simulink model "RobustFormationControl_FractionalModel_under_Dis"  (R2023a)
settings: Solver=ode3  StartTime=0.0  StopTime=30  FixedStep=0.0001  RelTol=1e-3
InitFcn:
  | % close all;
  | % clear all;
  | % clc;
  | % System & Qaudrotor Parameters
  | %==============================
  | m = 0.486;                                         % Quadrotor Mass ( kg )
  | 
  | L = 0.25;                                         % Length of the arm ( m )
  | % L = 0.25;                                         % Length of the arm ( m )
  | 
  | Ixx = 4.856e-03; Iyy = 4.856e-03; Izz = 8.801e-03; % The moments of inertia around x,y and z axes respectively ( kg.m^2 )
  | % Ixx = 3.8278e-03; Iyy = 3.8278e-03; Izz = 7.6566e-03; % The moments of inertia around x,y and z axes respectively ( kg.m^2 )
  | 
  | Jr = 2.8385e-5;                                            % The inertia moment of rotor ( kg.m^2 )
  | % Jr = 0;
  | 
  | % Kx=5.5670e-4;
  | % Ky=5.5670e-4;
  | % Kz=6.3540e-4;
  | % kx=0.032;
  | % ky=0.032;
  | % kz=0.048;
  | Kfx = 5.5670e-4; Kfy = 5.5670e-4; Kfz = 6.3540e-4;% The Rotational drag cofficients ( N/rad/s )
  | 
  | % Ktx = 0.032; Kty = 0.032; Ktz = 0.048;               % The linear drag coefficients in x, y, z respectively ( N/m/s )
  | Ktx = 5.5670e-4; Kty =5.5670e-4; Ktz = 6.3540e-4;               % The linear drag coefficients in x, y, z respectively ( N/m/s )
  | 
  | b = 2.923e-05;                                      % The lift coefficient
  | % b = 2.9842e-05;                                      % The lift coefficient
  | 
  | d = 1.12e-06;                                       % The drag coefficient
  | % d = 3.2320e-07;                                       % The drag coefficient
  | 
  | g = 9.81;                                          % The acceleration due to gravity ( m/s^2 )
  | 
  | %-------- The Coefficients of Non-linear Equations of Quadrotor ( Page 11) -------
  | %--------------------------------------------------------------------------------
  | % Rotational Equations
  | %=====================
  | % Coefficients in ( eq1 ) >>..
  | a1 = (Iyy - Izz)/Ixx;
  | b1 = - Jr/Ixx;
  | c1 = - Kfx/Ixx;
  | d1 = L/Ixx;
  | 
  | % Coefficients in ( eq2 ) >>..
  | a2 = (Izz - Ixx)/Iyy;
  | b2 = Jr/Iyy;
  | c2 = - Kfy/Iyy;
  | d2 = L/Iyy;
  | 
  | % Coefficients in ( eq3 ) >>..
  | a3 = (Ixx - Iyy)/Izz;
  | b3 = - Kfz/Izz;
  | c3 = 1/Izz;
  | % c3 = d/Izz;
  | 
  | % Translational Equations
  | %========================
  | % Coefficients in ( eq4 ) >>..
  | ... (+151 lines)
libraries: fod x135, eeStairGenerator x5
(part 10 of 10)

== system RobustFormationControl_FractionalModel_under_Dis/Fractional Leader with four followers/Fractional Model of the Leader/Fractional Model/Control Module1/Desired System/Desired Values/Helical Trajectry1 ==
  t : Inport
  Constant : Constant  Value=-1
  Gain : Gain  Gain=dis
  Gain1 : Gain  Gain=2*pi/15
  Gain2 : Gain  Gain=1/15
  Gain3 : Gain  Gain=2*pi/15
  Scope : Scope
  Step : Step  Time=0  After=0  SampleTime=0.03
  Step1 : Step  Time=0  SampleTime=0
  Step2 : Step  Time=5  After=0.5  SampleTime=0.03
  Step3 : Step  Time=10  After=0.5  SampleTime=0.03
  Sum : Sum  Inputs=++-
  Sum1 : Sum  Inputs=|+++
  Trigonometric Function : Trigonometry  Operator=cos
  Trigonometric Function1 : Trigonometry
  xd : Outport  VectorParamsAs1DForOutWhenUnconnected=off
  yd : Outport  Port=2  VectorParamsAs1DForOutWhenUnconnected=off
  zd : Outport  Port=3  VectorParamsAs1DForOutWhenUnconnected=off
  Psi_d : Outport  Port=4  VectorParamsAs1DForOutWhenUnconnected=off
  wires:
  t/1 -> Gain1/1, Gain3/1, Gain2/1
  Gain2/1 -> zd/1
  Step1/1 -> Psi_d/1
  Trigonometric Function1/1 -> yd/1
  Step/1 -> Sum/1
  Sum/1 -> Gain/1, Scope/1
  Step2/1 -> Sum/2
  Step3/1 -> Sum/3
  Sum1/1 -> xd/1
  Trigonometric Function/1 -> Sum1/2
  Gain/1 -> Sum1/1
  Gain1/1 -> Trigonometric Function/1
  Gain3/1 -> Trigonometric Function1/1
  Constant/1 -> Sum1/3

== system RobustFormationControl_FractionalModel_under_Dis/Fractional Leader with four followers/Fractional Model of the Leader/Fractional Model/Control Module1/Desired System/Desired Values/Step Inputs Trajectry ==
  Step : Step  Time=0  After=3  SampleTime=0
  Step1 : Step  Time=0  After=5  SampleTime=0
  Step2 : Step  Time=0  SampleTime=0
  Step3 : Step  Time=0  After=2  SampleTime=0
  xd : Outport  VectorParamsAs1DForOutWhenUnconnected=off
  yd : Outport  Port=2  VectorParamsAs1DForOutWhenUnconnected=off
  zd : Outport  Port=3  VectorParamsAs1DForOutWhenUnconnected=off
  Psi_d : Outport  Port=4  VectorParamsAs1DForOutWhenUnconnected=off
  wires:
  Step2/1 -> xd/1
  Step3/1 -> yd/1
  Step/1 -> zd/1
  Step1/1 -> Psi_d/1

== matlab function RobustFormationControl_FractionalModel_under_Dis/Fractional Leader with four followers/Fractional Model of the Leader/Stochastic Disturbances/Dphi2/MATLAB Function ==
  data: t input; Dphi2 output
function Dphi2 = fcn(t)

Dphi2 = 0.5*cos(0.5*t) + 1;

== matlab function RobustFormationControl_FractionalModel_under_Dis/Fractional Leader with four followers/Fractional Model of the Leader/Stochastic Disturbances/Dphi3/MATLAB Function ==
  data: t input; Dphi3 output
function Dphi3 = fcn(t)

Dphi3 = 0.05*cos(0.7*t) + 0.1;

== matlab function RobustFormationControl_FractionalModel_under_Dis/Fractional Leader with four followers/Fractional Model of the Leader/Stochastic Disturbances/Dpx/MATLAB Function ==
  data: t input; Dpx output
function Dpx = fcn(t)

Dpx = -0.08*sin(0.11*t - 3.0403) + 0.04*sin(0.5*t - 13.5) + 0.008*sin(1.6*t -15*pi) +0.006*sin(0.3*t - 8.6);

== matlab function RobustFormationControl_FractionalModel_under_Dis/Fractional Leader with four followers/Fractional Model of the Leader/Stochastic Disturbances/Dpy/MATLAB Function ==
  data: t input; Dpy output
function Dpy = fcn(t)

Dpy = 0.05*sin(0.4*t) + 0.05*cos(0.7*t);

== matlab function RobustFormationControl_FractionalModel_under_Dis/Fractional Leader with four followers/Fractional Model of the Leader/Stochastic Disturbances/Dpz/MATLAB Function ==
  data: t input; Dpz output
function Dpz = fcn(t)

Dpz = 0.05*sin(0.7*t) + 0.07*cos(0.3*t);

== matlab function RobustFormationControl_FractionalModel_under_Dis/Fractional Leader with four followers/Fractional Model of the Leader/Stochastic Disturbances/Dphi1/MATLAB Function ==
  data: t input; Dphi1 output
function Dphi1 = fcn(t)

Dphi1 = 0.5*cos(0.4*t) + 1;
